simulink model "s_c107m32k_vlbi"  (R2018a)
settings: Solver=VariableStepDiscrete  StartTime=0.0  StopTime=(2^15)*10  RelTol=1e-3
undefined symbols (not defined in the file): fft_stages, n_bits_xengs
libraries: xbsIndex_r4 x23049, casper_library_misc x45, xps_library x4, casper_library_scopes x3, simulink x2
(part 29 of 201)

== system s_c107m32k_vlbi/quant_snap_filter1 ==
  note: This block filters out a single channel
      | from the quantiser so that if you want to get
      | a time-series of them in the snap instead of
      | a spectrum, you can do so.
  sync_in : Inport
  data_valid_in : Inport  Port=2
  data_in : Inport  Port=3
  packet_sync_in : Inport  Port=4
  single_channel_enable : Inport  Port=5
  channel_select : Inport  Port=6
  AddSub : xbsIndex_r4/AddSub  mode=Addition  use_carryin=off  use_carryout=off  en=off  latency=0  precision=User Defined  arith_type=Unsigned  n_bits=16  bin_pt=0  quantization=Truncate  overflow=Wrap  use_behavioral_HDL=off  hw_selection=Fabric  pipelined=off  dbl_ovrd=off  block_type=addsub
  Constant : xbsIndex_r4/Constant  const=4  gui_display_data_type=Fixed-point  arith_type=Unsigned  n_bits=3  bin_pt=0  preci_type=Single  exp_width=8  frac_width=24  explicit_period=on  period=1  equ=P=C  opselect=C  inp2=PCIN>>17  opr=+  inp1=P  carry=CIN  dbl_ovrd=off  block_type=constant
  Constant1 : xbsIndex_r4/Constant  const=0  gui_display_data_type=Fixed-point  arith_type=Unsigned  n_bits=3  bin_pt=0  preci_type=Single  exp_width=8  frac_width=24  explicit_period=on  period=1  equ=P=C  opselect=C  inp2=PCIN>>17  opr=+  inp1=P  carry=CIN  dbl_ovrd=off  block_type=constant
  Counter : xbsIndex_r4/Counter  cnt_type=Free Running  cnt_to=4095  operation=Up  start_count=0  cnt_by_val=4  arith_type=Unsigned  n_bits=fft_stages - 1  bin_pt=0  load_pin=off  rst=on  en=on  explicit_period=on  period=1  use_behavioral_HDL=off  implementation=Fabric  dbl_ovrd=off  block_type=counter
  Delay : xbsIndex_r4/Delay  rst=off  infoeditControl=Selection of Reset will increase slice count due to use of real FFs and instead of SRLs  en=off  latency=3  reg_retiming=off  dbl_ovrd=off  block_type=delay
  Delay{1..2,11..13} (5 alike) : xbsIndex_r4/Delay  rst=off  infoeditControl=Selection of Reset will increase slice count due to use of real FFs and instead of SRLs  en=off  latency=1  reg_retiming=off  dbl_ovrd=off  block_type=delay
  Delay{5,8..10} (4 alike) : xbsIndex_r4/Delay  rst=off  infoeditControl=Selection of Reset will increase slice count due to use of real FFs and instead of SRLs  en=off  latency=2  reg_retiming=off  dbl_ovrd=off  block_type=delay
  Logical1 : xbsIndex_r4/Logical  logical_function=AND  inputs=4  en=off  latency=0  precision=Full  arith_type=Unsigned  n_bits=16  bin_pt=0  align_bp=on  dbl_ovrd=off  block_type=logical
  Mux1 : xbsIndex_r4/Mux  inputs=2  en=off  latency=3  precision=Full  arith_type=Unsigned  n_bits=16  bin_pt=14  quantization=Truncate  overflow=Wrap  dbl_ovrd=off  block_type=mux
  Mux2 : xbsIndex_r4/Mux  inputs=2  en=off  latency=3  precision=Full  arith_type=Unsigned  n_bits=16  bin_pt=14  quantization=Truncate  overflow=Wrap  dbl_ovrd=off  block_type=mux
  Register : xbsIndex_r4/Register  init=0  rst=on  en=on  dbl_ovrd=off  block_type=register
  Register1 : xbsIndex_r4/Register  init=0  rst=on  en=on  dbl_ovrd=off  block_type=register
  Relational1 : xbsIndex_r4/Relational  mode=a>=b  op_type=Bool  en=off  latency=2  dbl_ovrd=off  block_type=relational
  Relational2 : xbsIndex_r4/Relational  mode=a<b  op_type=Bool  en=off  latency=2  dbl_ovrd=off  block_type=relational
  Relational3 : xbsIndex_r4/Relational  mode=a=b  op_type=Bool  en=off  latency=1  dbl_ovrd=off  block_type=relational
  edge_detect1 : Subsystem  mask(edge_detect){edge=Rising, polarity=Active High, x_in=[0 0.08 0.08 0.16 0.16 0.24 0.24 0.32 0.32 0.4], y_in=[-1 -1  1  1  1  1  1  1  1  1], x_out=[0.6 0.68 0.68 0.76 0.76 0.84 0.84 0.92 0.92 1], y_out=[-1 -1  1  1 -1 -1 -1 -1 -1 -1]}
      mask prompts: edge "Edge Type"; polarity "Output Polarity"; x_in "Input X Positions"; y_in "Input Y Positions"; x_out "Output X Positions"; y_out "Output Y Positions"
      mask help: Output is active for one-cycle after each edge of the specified type (i.e. rising, falling or both).
      mask init: same as s_c107m32k_vlbi/edge_detect1
      settings: AttributesFormatString=|
      | rising edges
      | active high
      mask Help: Output is active for one-cycle after each edge of the specified type (i.e. rising, falling, or both).  Latency is zero.
      mask TypeOptions edge: Rising | Falling | Both
      mask TypeOptions polarity: Active High | Active Low
      mask Display:
      | plot(x_in_num,0.5+y_in_num*0.2);
      | plot(x_out_num,0.5+y_out_num*0.2);
  edge_detect2 : Subsystem  mask(edge_detect){edge=Rising, polarity=Active High, x_in=[0 0.08 0.08 0.16 0.16 0.24 0.24 0.32 0.32 0.4], y_in=[-1 -1  1  1  1  1  1  1  1  1], x_out=[0.6 0.68 0.68 0.76 0.76 0.84 0.84 0.92 0.92 1], y_out=[-1 -1  1  1 -1 -1 -1 -1 -1 -1]}
      mask prompts: edge "Edge Type"; polarity "Output Polarity"; x_in "Input X Positions"; y_in "Input Y Positions"; x_out "Output X Positions"; y_out "Output Y Positions"
      mask help: Output is active for one-cycle after each edge of the specified type (i.e. rising, falling or both).
      mask init: same as s_c107m32k_vlbi/edge_detect1
      settings: AttributesFormatString=|
      | rising edges
      | active high
      mask Help: Output is active for one-cycle after each edge of the specified type (i.e. rising, falling, or both).  Latency is zero.
      mask TypeOptions edge: Rising | Falling | Both
      mask TypeOptions polarity: Active High | Active Low
      mask Display:
      | plot(x_in_num,0.5+y_in_num*0.2);
      | plot(x_out_num,0.5+y_out_num*0.2);
  edge_detect9 : Subsystem  mask(edge_detect){edge=Rising, polarity=Active High, x_in=[0 0.08 0.08 0.16 0.16 0.24 0.24 0.32 0.32 0.4], y_in=[-1 -1  1  1  1  1  1  1  1  1], x_out=[0.6 0.68 0.68 0.76 0.76 0.84 0.84 0.92 0.92 1], y_out=[-1 -1  1  1 -1 -1 -1 -1 -1 -1]}
      mask prompts: edge "Edge Type"; polarity "Output Polarity"; x_in "Input X Positions"; y_in "Input Y Positions"; x_out "Output X Positions"; y_out "Output Y Positions"
      mask help: Output is active for one-cycle after each edge of the specified type (i.e. rising, falling or both).
      mask init: same as s_c107m32k_vlbi/edge_detect1
      settings: AttributesFormatString=|
      | rising edges
      | active high
      mask Help: Output is active for one-cycle after each edge of the specified type (i.e. rising, falling, or both).  Latency is zero.
      mask TypeOptions edge: Rising | Falling | Both
      mask TypeOptions polarity: Active High | Active Low
      mask Display:
      | plot(x_in_num,0.5+y_in_num*0.2);
      | plot(x_out_num,0.5+y_out_num*0.2);
  data_valid_out : Outport
  data_out : Outport  Port=2
  packet_sync_out : Outport  Port=3
  wires:
  Delay13/1 -> Delay9/1
  Delay12/1 -> Delay8/1
  Delay11/1 -> Delay10/1, Delay2/1
  [packet_sync] -> Register1/3, Register1/1
  [sync_in] -> Register1/2
  Register1/1 -> edge_detect2/1(in)
  edge_detect2/1(out) -> Counter/1, Register/2
  Delay10/1 -> Mux2/2
  Delay9/1 -> Mux1/2
  Delay8/1 -> Delay/1
  edge_detect1/1(out) -> [selected_channel_active]
  edge_detect9/1(out) -> Mux2/3
  Logical1/1 -> edge_detect1/1(in)
  Delay5/1 -> Logical1/4
  Relational1/1 -> Logical1/3
  Relational2/1 -> Logical1/2
  Constant1/1 -> Relational3/1
  Relational3/1 -> edge_detect9/1(in)
  Counter/1 -> Relational3/2, AddSub/2, Relational1/2
  Delay2/1 -> Register/1, Register/3
  Register/1 -> Logical1/1
  AddSub/1 -> Relational2/2
  Constant/1 -> AddSub/1
  [packet_sync] -> Delay11/1
  Delay/1 -> data_out/1
  data_valid_in/1 -> [data_valid]
  Mux1/1 -> data_valid_out/1
  data_in/1 -> [data]
  [data_valid] -> Delay13/1
  sync_in/1 -> [sync_in]
  [selected_channel_active] -> Mux1/3
  packet_sync_in/1 -> [packet_sync]
  [data] -> Delay12/1
  [channel_select] -> Relational1/1, Relational2/1
  Mux2/1 -> packet_sync_out/1
  single_channel_enable/1 -> [single_channel_enable]
  [data_valid] -> Delay1/1
  [single_channel_enable] -> Mux1/1, Mux2/1
  channel_select/1 -> [channel_select]
  Delay1/1 -> Counter/2, Delay5/1

== system s_c107m32k_vlbi/quant_status ==
  out_pol0_or_cnt : Inport
  out_pol1_or_cnt : Inport  Port=2
  assert_pol0_or_cnt : xbsIndex_r4/Assert  assert_type=on  type_source=Explicitly  gui_display_data_type=Fixed-point  arith_type=Unsigned  n_bits=6  bin_pt=0  preci_type=Single  exp_width=8  frac_width=24  assert_rate=off  rate_source=Explicitly  period=1  output_port=on  block_type=assert
  assert_pol1_or_cnt : xbsIndex_r4/Assert  assert_type=on  type_source=Explicitly  gui_display_data_type=Fixed-point  arith_type=Unsigned  n_bits=6  bin_pt=0  preci_type=Single  exp_width=8  frac_width=24  assert_rate=off  rate_source=Explicitly  period=1  output_port=on  block_type=assert
  cast_gw : xbsIndex_r4/Convert  gui_display_data_type=Fixed-point  arith_type=Unsigned  n_bits=32  bin_pt=0  float_type=Single  exp_bits=8  fraction_bits=24  quantization=Truncate  overflow=Wrap  en=off  latency=1  pipeline=off  dbl_ovrd=off  block_type=convert
  concatenate : xbsIndex_r4/Concat  num_inputs=2  dbl_ovrd=off  block_type=concat
  io_delay : xbsIndex_r4/Delay  rst=off  infoeditControl=Selection of Reset will increase slice count due to use of real FFs and instead of SRLs  en=off  latency=0  reg_retiming=on  dbl_ovrd=off  block_type=delay
  reint1 : xbsIndex_r4/Reinterpret  force_arith_type=on  arith_type=Unsigned  force_bin_pt=on  bin_pt=0  block_type=reinterpret
  reint2 : xbsIndex_r4/Reinterpret  force_arith_type=on  arith_type=Unsigned  force_bin_pt=on  bin_pt=0  block_type=reinterpret
  s_c107m32k_vlbi_quant_status_user_data_in : xbsIndex_r4/Gateway Out  inherit_from_input=off  hdl_port=on  rows=1  columns=1  UseAsDAC=off  DACChannel='1'  interface=None  automatic_assignment=on  address_offset=hex2dec('00')  intf_name=''  intf_description=''  timing_constraint=None  locs_specified=off  LOCs={}  io_standard={}  block_type=gatewayout
  sim_out : Terminator
  wires:
  concatenate/1 -> io_delay/1
  io_delay/1 -> cast_gw/1
  cast_gw/1 -> s_c107m32k_vlbi_quant_status_user_data_in/1
  s_c107m32k_vlbi_quant_status_user_data_in/1 -> sim_out/1
  out_pol0_or_cnt/1 -> assert_pol0_or_cnt/1
  assert_pol0_or_cnt/1 -> reint1/1
  reint1/1 -> concatenate/1
  out_pol1_or_cnt/1 -> assert_pol1_or_cnt/1
  assert_pol1_or_cnt/1 -> reint2/1
  reint2/1 -> concatenate/2

== system s_c107m32k_vlbi/quant_sync_cnt ==
  out_reg : Inport
  assert_reg : xbsIndex_r4/Assert  assert_type=on  type_source=Explicitly  gui_display_data_type=Fixed-point  arith_type=Unsigned  n_bits=11  bin_pt=0  preci_type=Single  exp_width=8  frac_width=24  assert_rate=off  rate_source=Explicitly  period=1  output_port=on  block_type=assert
  cast_gw : xbsIndex_r4/Convert  gui_display_data_type=Fixed-point  arith_type=Unsigned  n_bits=32  bin_pt=0  float_type=Single  exp_bits=8  fraction_bits=24  quantization=Truncate  overflow=Wrap  en=off  latency=1  pipeline=off  dbl_ovrd=off  block_type=convert
  io_delay : xbsIndex_r4/Delay  rst=off  infoeditControl=Selection of Reset will increase slice count due to use of real FFs and instead of SRLs  en=off  latency=0  reg_retiming=on  dbl_ovrd=off  block_type=delay
  reint1 : xbsIndex_r4/Reinterpret  force_arith_type=on  arith_type=Unsigned  force_bin_pt=on  bin_pt=0  block_type=reinterpret
  s_c107m32k_vlbi_quant_sync_cnt_user_data_in : xbsIndex_r4/Gateway Out  inherit_from_input=off  hdl_port=on  rows=1  columns=1  UseAsDAC=off  DACChannel='1'  interface=None  automatic_assignment=on  address_offset=hex2dec('00')  intf_name=''  intf_description=''  timing_constraint=None  locs_specified=off  LOCs={}  io_standard={}  block_type=gatewayout
  sim_out : Terminator
  wires:
  io_delay/1 -> cast_gw/1
  cast_gw/1 -> s_c107m32k_vlbi_quant_sync_cnt_user_data_in/1
  s_c107m32k_vlbi_quant_sync_cnt_user_data_in/1 -> sim_out/1
  out_reg/1 -> assert_reg/1
  assert_reg/1 -> reint1/1
  reint1/1 -> io_delay/1

== system s_c107m32k_vlbi/reorder_status ==
  out_timestep_err_cnt : Inport
  out_receive_err_cnt : Inport  Port=2
  out_discard_cnt : Inport  Port=3
  out_relock_err_cnt : Inport  Port=4
  out_overflow_err_cnt : Inport  Port=5
  out_dv_cnt : Inport  Port=6
  assert_discard_cnt : xbsIndex_r4/Assert  assert_type=on  type_source=Explicitly  gui_display_data_type=Fixed-point  arith_type=Unsigned  n_bits=5  bin_pt=0  preci_type=Single  exp_width=8  frac_width=24  assert_rate=off  rate_source=Explicitly  period=1  output_port=on  block_type=assert
  assert_dv_cnt : xbsIndex_r4/Assert  assert_type=on  type_source=Explicitly  gui_display_data_type=Fixed-point  arith_type=Unsigned  n_bits=5  bin_pt=0  preci_type=Single  exp_width=8  frac_width=24  assert_rate=off  rate_source=Explicitly  period=1  output_port=on  block_type=assert
  assert_overflow_err_cnt : xbsIndex_r4/Assert  assert_type=on  type_source=Explicitly  gui_display_data_type=Fixed-point  arith_type=Unsigned  n_bits=5  bin_pt=0  preci_type=Single  exp_width=8  frac_width=24  assert_rate=off  rate_source=Explicitly  period=1  output_port=on  block_type=assert
  assert_receive_err_cnt : xbsIndex_r4/Assert  assert_type=on  type_source=Explicitly  gui_display_data_type=Fixed-point  arith_type=Unsigned  n_bits=5  bin_pt=0  preci_type=Single  exp_width=8  frac_width=24  assert_rate=off  rate_source=Explicitly  period=1  output_port=on  block_type=assert
  assert_relock_err_cnt : xbsIndex_r4/Assert  assert_type=on  type_source=Explicitly  gui_display_data_type=Fixed-point  arith_type=Unsigned  n_bits=5  bin_pt=0  preci_type=Single  exp_width=8  frac_width=24  assert_rate=off  rate_source=Explicitly  period=1  output_port=on  block_type=assert
  assert_timestep_err_cnt : xbsIndex_r4/Assert  assert_type=on  type_source=Explicitly  gui_display_data_type=Fixed-point  arith_type=Unsigned  n_bits=5  bin_pt=0  preci_type=Single  exp_width=8  frac_width=24  assert_rate=off  rate_source=Explicitly  period=1  output_port=on  block_type=assert
  cast_gw : xbsIndex_r4/Convert  gui_display_data_type=Fixed-point  arith_type=Unsigned  n_bits=32  bin_pt=0  float_type=Single  exp_bits=8  fraction_bits=24  quantization=Truncate  overflow=Wrap  en=off  latency=1  pipeline=off  dbl_ovrd=off  block_type=convert
  concatenate : xbsIndex_r4/Concat  num_inputs=6  dbl_ovrd=off  block_type=concat
  io_delay : xbsIndex_r4/Delay  rst=off  infoeditControl=Selection of Reset will increase slice count due to use of real FFs and instead of SRLs  en=off  latency=0  reg_retiming=on  dbl_ovrd=off  block_type=delay
  reint{1..6} (6 alike) : xbsIndex_r4/Reinterpret  force_arith_type=on  arith_type=Unsigned  force_bin_pt=on  bin_pt=0  block_type=reinterpret
  s_c107m32k_vlbi_reorder_status_user_data_in : xbsIndex_r4/Gateway Out  inherit_from_input=off  hdl_port=on  rows=1  columns=1  UseAsDAC=off  DACChannel='1'  interface=None  automatic_assignment=on  address_offset=hex2dec('00')  intf_name=''  intf_description=''  timing_constraint=None  locs_specified=off  LOCs={}  io_standard={}  block_type=gatewayout
  sim_out : Terminator
  wires:
  concatenate/1 -> io_delay/1
  io_delay/1 -> cast_gw/1
  cast_gw/1 -> s_c107m32k_vlbi_reorder_status_user_data_in/1
  s_c107m32k_vlbi_reorder_status_user_data_in/1 -> sim_out/1
  out_timestep_err_cnt/1 -> assert_timestep_err_cnt/1
  assert_timestep_err_cnt/1 -> reint1/1
  reint1/1 -> concatenate/1
  out_receive_err_cnt/1 -> assert_receive_err_cnt/1
  assert_receive_err_cnt/1 -> reint2/1
  reint2/1 -> concatenate/2
  out_discard_cnt/1 -> assert_discard_cnt/1
  assert_discard_cnt/1 -> reint3/1
  reint3/1 -> concatenate/3
  out_relock_err_cnt/1 -> assert_relock_err_cnt/1
  assert_relock_err_cnt/1 -> reint4/1
  reint4/1 -> concatenate/4
  out_overflow_err_cnt/1 -> assert_overflow_err_cnt/1
  assert_overflow_err_cnt/1 -> reint5/1
  reint5/1 -> concatenate/5
  out_dv_cnt/1 -> assert_dv_cnt/1
  assert_dv_cnt/1 -> reint6/1
  reint6/1 -> concatenate/6

== system s_c107m32k_vlbi/reorder_status1 ==
  out_dv_per_sec : Inport
  assert_dv_per_sec : xbsIndex_r4/Assert  assert_type=on  type_source=Explicitly  gui_display_data_type=Fixed-point  arith_type=Unsigned  n_bits=32  bin_pt=0  preci_type=Single  exp_width=8  frac_width=24  assert_rate=off  rate_source=Explicitly  period=1  output_port=on  block_type=assert
  cast_gw : xbsIndex_r4/Convert  gui_display_data_type=Fixed-point  arith_type=Unsigned  n_bits=32  bin_pt=0  float_type=Single  exp_bits=8  fraction_bits=24  quantization=Truncate  overflow=Wrap  en=off  latency=1  pipeline=off  dbl_ovrd=off  block_type=convert
  io_delay : xbsIndex_r4/Delay  rst=off  infoeditControl=Selection of Reset will increase slice count due to use of real FFs and instead of SRLs  en=off  latency=0  reg_retiming=on  dbl_ovrd=off  block_type=delay
  reint1 : xbsIndex_r4/Reinterpret  force_arith_type=on  arith_type=Unsigned  force_bin_pt=on  bin_pt=0  block_type=reinterpret
  s_c107m32k_vlbi_reorder_status1_user_data_in : xbsIndex_r4/Gateway Out  inherit_from_input=off  hdl_port=on  rows=1  columns=1  UseAsDAC=off  DACChannel='1'  interface=None  automatic_assignment=on  address_offset=hex2dec('00')  intf_name=''  intf_description=''  timing_constraint=None  locs_specified=off  LOCs={}  io_standard={}  block_type=gatewayout
  sim_out : Terminator
  wires:
  io_delay/1 -> cast_gw/1
  cast_gw/1 -> s_c107m32k_vlbi_reorder_status1_user_data_in/1
  s_c107m32k_vlbi_reorder_status1_user_data_in/1 -> sim_out/1
  out_dv_per_sec/1 -> assert_dv_per_sec/1
  assert_dv_per_sec/1 -> reint1/1
  reint1/1 -> io_delay/1

== system s_c107m32k_vlbi/rx_dest_ip ==
  out_reg : Inport
  assert_reg : xbsIndex_r4/Assert  assert_type=on  type_source=Explicitly  gui_display_data_type=Fixed-point  arith_type=Unsigned  n_bits=32  bin_pt=0  preci_type=Single  exp_width=8  frac_width=24  assert_rate=off  rate_source=Explicitly  period=1  output_port=on  block_type=assert
  cast_gw : xbsIndex_r4/Convert  gui_display_data_type=Fixed-point  arith_type=Unsigned  n_bits=32  bin_pt=0  float_type=Single  exp_bits=8  fraction_bits=24  quantization=Truncate  overflow=Wrap  en=off  latency=1  pipeline=off  dbl_ovrd=off  block_type=convert
  io_delay : xbsIndex_r4/Delay  rst=off  infoeditControl=Selection of Reset will increase slice count due to use of real FFs and instead of SRLs  en=off  latency=0  reg_retiming=on  dbl_ovrd=off  block_type=delay
  reint1 : xbsIndex_r4/Reinterpret  force_arith_type=on  arith_type=Unsigned  force_bin_pt=on  bin_pt=0  block_type=reinterpret
  s_c107m32k_vlbi_rx_dest_ip_user_data_in : xbsIndex_r4/Gateway Out  inherit_from_input=off  hdl_port=on  rows=1  columns=1  UseAsDAC=off  DACChannel='1'  interface=None  automatic_assignment=on  address_offset=hex2dec('00')  intf_name=''  intf_description=''  timing_constraint=None  locs_specified=off  LOCs={}  io_standard={}  block_type=gatewayout
  sim_out : Terminator
  wires:
  io_delay/1 -> cast_gw/1
  cast_gw/1 -> s_c107m32k_vlbi_rx_dest_ip_user_data_in/1
  s_c107m32k_vlbi_rx_dest_ip_user_data_in/1 -> sim_out/1
  out_reg/1 -> assert_reg/1
  assert_reg/1 -> reint1/1
  reint1/1 -> io_delay/1

== system s_c107m32k_vlbi/simple_bram_vacc1 ==
  new_acc : Inport
  din : Inport  Port=2
  dvalid : Inport  Port=3
  Adder : xbsIndex_r4/AddSub  mode=Addition  use_carryin=off  use_carryout=off  en=on  latency=2  precision=User Defined  arith_type=Unsigned  n_bits=n_bits  bin_pt=bin_pt  quantization=Truncate  overflow=Wrap  use_behavioral_HDL=on  hw_selection=Fabric  pipelined=off  use_rpm=on  dbl_ovrd=off  block_type=addsub
      settings: xl_area=[0, 0, 0, 0, 0, 0, 0]  block_version=10.1.3
  Constant : xbsIndex_r4/Constant  const=0  gui_display_data_type=Fixed-point  arith_type=Unsigned  n_bits=n_bits  bin_pt=bin_pt  preci_type=Single  exp_width=8  frac_width=24  explicit_period=on  period=1  equ=P=C  opselect=C  inp2=PCIN>>17  opr=+  inp1=P  carry=CIN  dbl_ovrd=off  block_type=constant
  Delay17 : xbsIndex_r4/Delay  rst=off  infoeditControl=Selection of Reset will increase slice count due to use of real FFs and instead of SRLs  en=off  latency=1  reg_retiming=on  dbl_ovrd=off  block_type=delay
  Gateway Out{1..3,71} (4 alike) : xbsIndex_r4/Gateway Out  inherit_from_input=off  hdl_port=off  rows=1  columns=1  UseAsDAC=off  DACChannel='1'  interface=None  automatic_assignment=on  address_offset=hex2dec('00')  intf_name=''  intf_description=''  timing_constraint=None  locs_specified=off  LOCs={}  io_standard={}  block_type=gatewayout
  Logical : xbsIndex_r4/Logical  logical_function=AND  inputs=2  en=off  latency=0  precision=Full  arith_type=Unsigned  n_bits=16  bin_pt=0  align_bp=on  dbl_ovrd=off  block_type=logical
  Mux : xbsIndex_r4/Mux  inputs=2  en=off  latency=0  precision=Full  arith_type="Signed  (2's comp)"  n_bits=8  bin_pt=2  quantization=Truncate  overflow=Wrap  dbl_ovrd=off  block_type=mux
      settings: xl_area=[0, 0, 0, 0, 0, 0, 0]
  To Workspace1 : ToWorkspace  VariableName=tp28  SaveFormat=Timeseries  SampleTime=-1
  To Workspace2 : ToWorkspace  VariableName=tp29  SaveFormat=Timeseries  SampleTime=-1
  To Workspace3 : ToWorkspace  VariableName=tp30  SaveFormat=Timeseries  SampleTime=-1
  To Workspace71 : ToWorkspace  VariableName=tp27  SaveFormat=Timeseries  SampleTime=-1
  delay_bram : Subsystem  mask(delay_bram){DelayLen=vec_len - 2, bram_latency=2}
      mask prompts: DelayLen "Delay By:"; bram_latency "BRAM Latency"
      mask help: A delay block that uses BRAM for its storage.
      mask init:
      | if (DelayLen <= bram_latency)
      | 	error('delay value must be greater than BRAM Latency');
      | end
      | BitWidth = max(ceil(log2(DelayLen)), 2);
      mask Help: eval('xlWeb(''http://casper.berkeley.edu/wiki/Delay_bram'')')
  pulse_ext : Subsystem  mask(pulse_ext){pulse_len=vec_len}
      mask prompts: pulse_len "Length of Pulse"
      mask help:
      | Extends a boolean signal to be high for the specified number of clocks after
      | the last high input.
      mask init:
      | bits = ceil(log2(pulse_len+1));
      mask Help: eval('xlWeb(''http://casper.berkeley.edu/wiki/Pulse_ext'')')
  dout : Outport
  valid : Outport  Port=2
  wires:
  delay_bram/1(Out1) -> Gateway Out3/1, dout/1, Mux/2
  new_acc/1 -> pulse_ext/1(in)
  Constant/1 -> Mux/3
  din/1 -> Adder/1
  Adder/1 -> delay_bram/1(In1)
  pulse_ext/1(out) -> Gateway Out1/1, Logical/2, Mux/1
  dvalid/1 -> delay_bram/2(In2), Adder/3, Gateway Out71/1, Logical/1, pulse_ext/2(dvalid)
  Mux/1 -> Adder/2
  Logical/1 -> Delay17/1
  Gateway Out71/1 -> To Workspace71/1
  Gateway Out1/1 -> To Workspace1/1
  Gateway Out2/1 -> To Workspace2/1
  Gateway Out3/1 -> To Workspace3/1
  Delay17/1 -> Gateway Out2/1, valid/1

== system s_c107m32k_vlbi/simple_bram_vacc2 ==
  new_acc : Inport
  din : Inport  Port=2
  dvalid : Inport  Port=3
  Adder : xbsIndex_r4/AddSub  mode=Addition  use_carryin=off  use_carryout=off  en=on  latency=2  precision=User Defined  arith_type=Unsigned  n_bits=n_bits  bin_pt=bin_pt  quantization=Truncate  overflow=Wrap  use_behavioral_HDL=on  hw_selection=Fabric  pipelined=off  use_rpm=on  dbl_ovrd=off  block_type=addsub
      settings: xl_area=[0, 0, 0, 0, 0, 0, 0]  block_version=10.1.3
  Constant : xbsIndex_r4/Constant  const=0  gui_display_data_type=Fixed-point  arith_type=Unsigned  n_bits=n_bits  bin_pt=bin_pt  preci_type=Single  exp_width=8  frac_width=24  explicit_period=on  period=1  equ=P=C  opselect=C  inp2=PCIN>>17  opr=+  inp1=P  carry=CIN  dbl_ovrd=off  block_type=constant
  Delay17 : xbsIndex_r4/Delay  rst=off  infoeditControl=Selection of Reset will increase slice count due to use of real FFs and instead of SRLs  en=off  latency=2  reg_retiming=on  dbl_ovrd=off  block_type=delay
  Gateway Out{1..3,71} (4 alike) : xbsIndex_r4/Gateway Out  inherit_from_input=off  hdl_port=off  rows=1  columns=1  UseAsDAC=off  DACChannel='1'  interface=None  automatic_assignment=on  address_offset=hex2dec('00')  intf_name=''  intf_description=''  timing_constraint=None  locs_specified=off  LOCs={}  io_standard={}  block_type=gatewayout
  Logical : xbsIndex_r4/Logical  logical_function=AND  inputs=2  en=off  latency=0  precision=Full  arith_type=Unsigned  n_bits=16  bin_pt=0  align_bp=on  dbl_ovrd=off  block_type=logical
  Mux : xbsIndex_r4/Mux  inputs=2  en=off  latency=0  precision=Full  arith_type="Signed  (2's comp)"  n_bits=8  bin_pt=2  quantization=Truncate  overflow=Wrap  dbl_ovrd=off  block_type=mux
      settings: xl_area=[0, 0, 0, 0, 0, 0, 0]
  To Workspace1 : ToWorkspace  VariableName=tp28  SaveFormat=Timeseries  SampleTime=-1
  To Workspace2 : ToWorkspace  VariableName=tp29  SaveFormat=Timeseries  SampleTime=-1
  To Workspace3 : ToWorkspace  VariableName=tp30  SaveFormat=Timeseries  SampleTime=-1
  To Workspace71 : ToWorkspace  VariableName=tp27  SaveFormat=Timeseries  SampleTime=-1
  delay_bram : Subsystem  mask(delay_bram){DelayLen=vec_len - 2, bram_latency=2}
      mask prompts: DelayLen "Delay By:"; bram_latency "BRAM Latency"
      mask help: A delay block that uses BRAM for its storage.
      mask init:
      | if (DelayLen <= bram_latency)
      | 	error('delay value must be greater than BRAM Latency');
      | end
      | BitWidth = max(ceil(log2(DelayLen)), 2);
      mask Help: eval('xlWeb(''http://casper.berkeley.edu/wiki/Delay_bram'')')
  pulse_ext : Subsystem  mask(pulse_ext){pulse_len=vec_len}
      mask prompts: pulse_len "Length of Pulse"
      mask help:
      | Extends a boolean signal to be high for the specified number of clocks after
      | the last high input.
      mask init:
      | bits = ceil(log2(pulse_len+1));
      mask Help: eval('xlWeb(''http://casper.berkeley.edu/wiki/Pulse_ext'')')
  dout : Outport
  valid : Outport  Port=2
  wires:
  Delay17/1 -> valid/1, Gateway Out2/1
  Gateway Out3/1 -> To Workspace3/1
  Gateway Out2/1 -> To Workspace2/1
  Gateway Out1/1 -> To Workspace1/1
  Gateway Out71/1 -> To Workspace71/1
  Logical/1 -> Delay17/1
  Mux/1 -> Adder/2
  dvalid/1 -> pulse_ext/2(dvalid), Logical/1, Gateway Out71/1, Adder/3, delay_bram/2(In2)
  pulse_ext/1(out) -> Mux/1, Logical/2, Gateway Out1/1
  Adder/1 -> delay_bram/1(In1)
  din/1 -> Adder/1
  Constant/1 -> Mux/3
  new_acc/1 -> pulse_ext/1(in)
  delay_bram/1(Out1) -> Mux/2, dout/1, Gateway Out3/1

== system s_c107m32k_vlbi/snap_acc ==
  in_acc : Inport
  we : Inport  Port=2
  trig : Inport  Port=3
  assert_acc : xbsIndex_r4/Assert  assert_type=on  type_source=Explicitly  gui_display_data_type=Fixed-point  arith_type=Unsigned  n_bits=32  bin_pt=10  preci_type=Single  exp_width=8  frac_width=24  assert_rate=off  rate_source=Explicitly  period=1  output_port=on  block_type=assert
  buscreate : Subsystem  AncestorBlock=casper_library_flow_control/bus_create  mask(bus_create){inputNum=1}
      mask prompts: inputNum "Number of inputs:"
      mask init:
      | bus_create_init(gcb,...
      |     'inputNum', inputNum);
  io_delay : Subsystem  AncestorBlock=casper_library_delays/pipeline  mask(pipeline){csp_latency=2}
      mask prompts: csp_latency "Latency"
      mask help:
      | An explicitly laid-out delay line to avoid mapping to SRL16s
      | for use in pipelining to help achieve timing closure.
      mask init:
      | pipeline_init(gcb,'latency',csp_latency);
      settings: AttributesFormatString=Latency = %<latency>
      mask Display:
      | port_label('input', 1, 'd');
      | port_label('output', 1, 'q');
      | disp(['Z^-', num2str(csp_latency)]);
  ss : Subsystem  Tag=casper:snapshot  AncestorBlock=casper_library_scopes/snapshot  mask(snapshot){storage=bram, dram_dimm=2, dram_clock=250, nsamples=15, data_width=32, offset=off, circap=off, value=off, ext_arm=off, ext_circ=off, provide_outputs=off, use_dsp48=on}
      mask prompts: storage "Storage medium"; dram_dimm "DRAM dimm"; dram_clock "DRAM clock rate"; nsamples "Number of Samples (2^?)"; data_width "Data width"; offset "Start delay support"; circap "Circular capture support"; value "Extra value capture support"; ext_arm "External arm support"; ext_circ "External circular capture support"; provide_outputs "Provide outputs"; use_dsp48 "Use DSP48s to implement counters"
      mask help:
      | Standard snap block, but with the following optional extras;
      |  1) Optionally delay the fabric trigger by a user-specified number of valids.
      |  2) Capture continuously after a trigger until a stop pulse is received. Data is captured into BRAM continuously, with old data being overwritten until a stop command is received. Then stop capturing when memory is filled. This enables you to get some data before and some data after the stop pulse. Use the 'tr_en_cnt' register to determine where you are in your vector. 'Addr' register's MSb now indicates 'busy capturing'.
      |  3) Optionally capture a value on an input port to a register at the same time as the first data sample.
      |  4) Implement counters using DSP48Es to save resources.
      mask init:
      | snapshot_init(gcb, ...
      |     'storage', storage, ...
      |     'dram_dimm', dram_dimm, ...
      |     'dram_clock', dram_clock, ...
      |     'nsamples', nsamples, ...
      |     'data_width', data_width, ...
      |     'offset', offset, ...
      |     'circap', circap, ...
      |     'value', value, ...
      |     'ext_arm', ext_arm, ...
      |     'ext_circ', ext_circ, ...
      |     'provide_outputs', 'off', ...
      |     'use_dsp48', use_dsp48);
      settings: AttributesFormatString=|
      | 32 wide, 32768 deep
      | debugID: 110166481
      mask TypeOptions storage: bram | dram
      mask Callback storage: snapshot_callback();
      mask TypeOptions dram_dimm: 1 | 2 | 3 | 4
      mask TypeOptions dram_clock: 200 | 250 | 266 | 300 | 333
      mask TypeOptions data_width: 8 | 16 | 32 | 64 | 128
  trig_delay : Subsystem  AncestorBlock=casper_library_delays/pipeline  mask(pipeline){csp_latency=2}
      mask prompts: csp_latency "Latency"
      mask help:
      | An explicitly laid-out delay line to avoid mapping to SRL16s
      | for use in pipelining to help achieve timing closure.
      mask init:
      | pipeline_init(gcb,'latency',csp_latency);
      settings: AttributesFormatString=Latency = %<latency>
      mask Display:
      | port_label('input', 1, 'd');
      | port_label('output', 1, 'q');
      | disp(['Z^-', num2str(csp_latency)]);
  we_delay : Subsystem  AncestorBlock=casper_library_delays/pipeline  mask(pipeline){csp_latency=2}
      mask prompts: csp_latency "Latency"
      mask help:
      | An explicitly laid-out delay line to avoid mapping to SRL16s
      | for use in pipelining to help achieve timing closure.
      mask init:
      | pipeline_init(gcb,'latency',csp_latency);
      settings: AttributesFormatString=Latency = %<latency>
      mask Display:
      | port_label('input', 1, 'd');
      | port_label('output', 1, 'q');
      | disp(['Z^-', num2str(csp_latency)]);
  arm_out : Outport
  wires:
  ss/1(arm_out) -> arm_out/1
  buscreate/1(bus_out) -> io_delay/1(d)
  io_delay/1(q) -> ss/1(din)
  in_acc/1 -> assert_acc/1
  assert_acc/1 -> buscreate/1(in1)
  we/1 -> we_delay/1(d)
  we_delay/1(q) -> ss/2(we)
  trig/1 -> trig_delay/1(d)
  trig_delay/1(q) -> ss/3(trig)

== system s_c107m32k_vlbi/snap_adc0 ==
  in_p0_d0 : Inport
  in_p0_d1 : Inport  Port=2
  in_p0_d2 : Inport  Port=3
  in_p0_d3 : Inport  Port=4
  in_p0_d4 : Inport  Port=5
  in_p0_d5 : Inport  Port=6
  in_p0_d6 : Inport  Port=7
  in_p0_d7 : Inport  Port=8
  in_dv : Inport  Port=9
  in_sync : Inport  Port=10
  we : Inport  Port=11
  trig : Inport  Port=12
  stop : Inport  Port=13
  extra_timestamp : Inport  Port=14
  assert_dv : xbsIndex_r4/Assert  assert_type=on  type_source=Explicitly  gui_display_data_type=Boolean  arith_type=Boolean  n_bits=1  bin_pt=0  preci_type=Single  exp_width=8  frac_width=24  assert_rate=off  rate_source=Explicitly  period=1  output_port=on  block_type=assert
  assert_p0_d{0..7} (8 alike) : xbsIndex_r4/Assert  assert_type=on  type_source=Explicitly  gui_display_data_type=Fixed-point  arith_type="Signed  (2's comp)"  n_bits=10  bin_pt=9  preci_type=Single  exp_width=8  frac_width=24  assert_rate=off  rate_source=Explicitly  period=1  output_port=on  block_type=assert
  assert_sync : xbsIndex_r4/Assert  assert_type=on  type_source=Explicitly  gui_display_data_type=Boolean  arith_type=Boolean  n_bits=1  bin_pt=0  preci_type=Single  exp_width=8  frac_width=24  assert_rate=off  rate_source=Explicitly  period=1  output_port=on  block_type=assert
  assextra_timestamp : xbsIndex_r4/Assert  assert_type=on  type_source=Explicitly  gui_display_data_type=Fixed-point  arith_type=Unsigned  n_bits=32  bin_pt=0  preci_type=Single  exp_width=8  frac_width=24  assert_rate=off  rate_source=Explicitly  period=1  output_port=on  block_type=assert
  buscreate : Subsystem  AncestorBlock=casper_library_flow_control/bus_create  mask(bus_create){inputNum=10}
      mask prompts: inputNum "Number of inputs:"
      mask init:
      | bus_create_init(gcb,...
      |     'inputNum', inputNum);
  extra_delay : Subsystem  AncestorBlock=casper_library_delays/pipeline  mask(pipeline){csp_latency=2}
      mask prompts: csp_latency "Latency"
      mask help:
      | An explicitly laid-out delay line to avoid mapping to SRL16s
      | for use in pipelining to help achieve timing closure.
      mask init:
      | pipeline_init(gcb,'latency',csp_latency);
      settings: AttributesFormatString=Latency = %<latency>
      mask Display:
      | port_label('input', 1, 'd');
      | port_label('output', 1, 'q');
      | disp(['Z^-', num2str(csp_latency)]);
  extracast : xbsIndex_r4/Convert  gui_display_data_type=Fixed-point  arith_type=Unsigned  n_bits=32  bin_pt=0  float_type=Single  exp_bits=8  fraction_bits=24  quantization=Truncate  overflow=Wrap  en=off  latency=1  pipeline=off  dbl_ovrd=off  block_type=convert
  extracreate : Subsystem  AncestorBlock=casper_library_flow_control/bus_create  mask(bus_create){inputNum=1}
      mask prompts: inputNum "Number of inputs:"
      mask init:
      | bus_create_init(gcb,...
      |     'inputNum', inputNum);
  io_delay : Subsystem  AncestorBlock=casper_library_delays/pipeline  mask(pipeline){csp_latency=2}
      mask prompts: csp_latency "Latency"
      mask help:
      | An explicitly laid-out delay line to avoid mapping to SRL16s
      | for use in pipelining to help achieve timing closure.
      mask init:
      | pipeline_init(gcb,'latency',csp_latency);
      settings: AttributesFormatString=Latency = %<latency>
      mask Display:
      | port_label('input', 1, 'd');
      | port_label('output', 1, 'q');
      | disp(['Z^-', num2str(csp_latency)]);
  ss : Subsystem  Tag=casper:snapshot  AncestorBlock=casper_library_scopes/snapshot  mask(snapshot){storage=bram, dram_dimm=2, dram_clock=250, nsamples=8, data_width=128, offset=off, circap=on, value=on, ext_arm=off, ext_circ=off, provide_outputs=off, use_dsp48=on}
      mask prompts: storage "Storage medium"; dram_dimm "DRAM dimm"; dram_clock "DRAM clock rate"; nsamples "Number of Samples (2^?)"; data_width "Data width"; offset "Start delay support"; circap "Circular capture support"; value "Extra value capture support"; ext_arm "External arm support"; ext_circ "External circular capture support"; provide_outputs "Provide outputs"; use_dsp48 "Use DSP48s to implement counters"
      mask help:
      | Standard snap block, but with the following optional extras;
      |  1) Optionally delay the fabric trigger by a user-specified number of valids.
      |  2) Capture continuously after a trigger until a stop pulse is received. Data is captured into BRAM continuously, with old data being overwritten until a stop command is received. Then stop capturing when memory is filled. This enables you to get some data before and some data after the stop pulse. Use the 'tr_en_cnt' register to determine where you are in your vector. 'Addr' register's MSb now indicates 'busy capturing'.
      |  3) Optionally capture a value on an input port to a register at the same time as the first data sample.
      |  4) Implement counters using DSP48Es to save resources.
      mask init: same as s_c107m32k_vlbi/snap_acc/ss
      settings: AttributesFormatString=|
      | 128 wide, 256 deep
      | debugID: 56897180
      mask TypeOptions storage: bram | dram
      mask Callback storage: snapshot_callback();
      mask TypeOptions dram_dimm: 1 | 2 | 3 | 4
      mask TypeOptions dram_clock: 200 | 250 | 266 | 300 | 333
      mask TypeOptions data_width: 8 | 16 | 32 | 64 | 128
  stop_delay : Subsystem  AncestorBlock=casper_library_delays/pipeline  mask(pipeline){csp_latency=2}
      mask prompts: csp_latency "Latency"
      mask help:
      | An explicitly laid-out delay line to avoid mapping to SRL16s
      | for use in pipelining to help achieve timing closure.
      mask init:
      | pipeline_init(gcb,'latency',csp_latency);
      settings: AttributesFormatString=Latency = %<latency>
      mask Display:
      | port_label('input', 1, 'd');
      | port_label('output', 1, 'q');
      | disp(['Z^-', num2str(csp_latency)]);
  trig_delay : Subsystem  AncestorBlock=casper_library_delays/pipeline  mask(pipeline){csp_latency=2}
      mask prompts: csp_latency "Latency"
      mask help:
      | An explicitly laid-out delay line to avoid mapping to SRL16s
      | for use in pipelining to help achieve timing closure.
      mask init:
      | pipeline_init(gcb,'latency',csp_latency);
      settings: AttributesFormatString=Latency = %<latency>
      mask Display:
      | port_label('input', 1, 'd');
      | port_label('output', 1, 'q');
      | disp(['Z^-', num2str(csp_latency)]);
  we_delay : Subsystem  AncestorBlock=casper_library_delays/pipeline  mask(pipeline){csp_latency=2}
      mask prompts: csp_latency "Latency"
      mask help:
      | An explicitly laid-out delay line to avoid mapping to SRL16s
      | for use in pipelining to help achieve timing closure.
      mask init:
      | pipeline_init(gcb,'latency',csp_latency);
      settings: AttributesFormatString=Latency = %<latency>
      mask Display:
      | port_label('input', 1, 'd');
      | port_label('output', 1, 'q');
      | disp(['Z^-', num2str(csp_latency)]);
  arm_out : Outport
  wires:
  ss/1(arm_out) -> arm_out/1
  buscreate/1(bus_out) -> io_delay/1(d)
  io_delay/1(q) -> ss/1(din)
  in_p0_d0/1 -> assert_p0_d0/1
  assert_p0_d0/1 -> buscreate/1(in1)
  in_p0_d1/1 -> assert_p0_d1/1
  assert_p0_d1/1 -> buscreate/2(in2)
  in_p0_d2/1 -> assert_p0_d2/1
  assert_p0_d2/1 -> buscreate/3(in3)
  in_p0_d3/1 -> assert_p0_d3/1
  assert_p0_d3/1 -> buscreate/4(in4)
  in_p0_d4/1 -> assert_p0_d4/1
  assert_p0_d4/1 -> buscreate/5(in5)
  in_p0_d5/1 -> assert_p0_d5/1
  assert_p0_d5/1 -> buscreate/6(in6)
  in_p0_d6/1 -> assert_p0_d6/1
  assert_p0_d6/1 -> buscreate/7(in7)
  in_p0_d7/1 -> assert_p0_d7/1
  assert_p0_d7/1 -> buscreate/8(in8)
  in_dv/1 -> assert_dv/1
  assert_dv/1 -> buscreate/9(in9)
  in_sync/1 -> assert_sync/1
  assert_sync/1 -> buscreate/10(in10)
  we/1 -> we_delay/1(d)
  we_delay/1(q) -> ss/2(we)
  trig/1 -> trig_delay/1(d)
  trig_delay/1(q) -> ss/3(trig)
  stop/1 -> stop_delay/1(d)
  stop_delay/1(q) -> ss/4(stop)
  extracreate/1(bus_out) -> extra_delay/1(d)
  extra_delay/1(q) -> extracast/1
  extracast/1 -> ss/5(vin)
  extra_timestamp/1 -> assextra_timestamp/1
  assextra_timestamp/1 -> extracreate/1(in1)

== system s_c107m32k_vlbi/snap_adc1 ==
  in_p1_d0 : Inport
  in_p1_d1 : Inport  Port=2
  in_p1_d2 : Inport  Port=3
  in_p1_d3 : Inport  Port=4
  in_p1_d4 : Inport  Port=5
  in_p1_d5 : Inport  Port=6
  in_p1_d6 : Inport  Port=7
  in_p1_d7 : Inport  Port=8
  we : Inport  Port=9
  trig : Inport  Port=10
  stop : Inport  Port=11
  extra_timestamp : Inport  Port=12
  assert_p1_d{0..7} (8 alike) : xbsIndex_r4/Assert  assert_type=on  type_source=Explicitly  gui_display_data_type=Fixed-point  arith_type="Signed  (2's comp)"  n_bits=10  bin_pt=9  preci_type=Single  exp_width=8  frac_width=24  assert_rate=off  rate_source=Explicitly  period=1  output_port=on  block_type=assert
  assextra_timestamp : xbsIndex_r4/Assert  assert_type=on  type_source=Explicitly  gui_display_data_type=Fixed-point  arith_type=Unsigned  n_bits=32  bin_pt=0  preci_type=Single  exp_width=8  frac_width=24  assert_rate=off  rate_source=Explicitly  period=1  output_port=on  block_type=assert
  buscreate : Subsystem  AncestorBlock=casper_library_flow_control/bus_create  mask(bus_create){inputNum=8}
      mask prompts: inputNum "Number of inputs:"
      mask init:
      | bus_create_init(gcb,...
      |     'inputNum', inputNum);
  extra_delay : Subsystem  AncestorBlock=casper_library_delays/pipeline  mask(pipeline){csp_latency=2}
      mask prompts: csp_latency "Latency"
      mask help:
      | An explicitly laid-out delay line to avoid mapping to SRL16s
      | for use in pipelining to help achieve timing closure.
      mask init:
      | pipeline_init(gcb,'latency',csp_latency);
      settings: AttributesFormatString=Latency = %<latency>
      mask Display:
      | port_label('input', 1, 'd');
      | port_label('output', 1, 'q');
      | disp(['Z^-', num2str(csp_latency)]);
  extracast : xbsIndex_r4/Convert  gui_display_data_type=Fixed-point  arith_type=Unsigned  n_bits=32  bin_pt=0  float_type=Single  exp_bits=8  fraction_bits=24  quantization=Truncate  overflow=Wrap  en=off  latency=1  pipeline=off  dbl_ovrd=off  block_type=convert
  extracreate : Subsystem  AncestorBlock=casper_library_flow_control/bus_create  mask(bus_create){inputNum=1}
      mask prompts: inputNum "Number of inputs:"
      mask init:
      | bus_create_init(gcb,...
      |     'inputNum', inputNum);
  io_delay : Subsystem  AncestorBlock=casper_library_delays/pipeline  mask(pipeline){csp_latency=2}
      mask prompts: csp_latency "Latency"
      mask help:
      | An explicitly laid-out delay line to avoid mapping to SRL16s
      | for use in pipelining to help achieve timing closure.
      mask init:
      | pipeline_init(gcb,'latency',csp_latency);
      settings: AttributesFormatString=Latency = %<latency>
      mask Display:
      | port_label('input', 1, 'd');
      | port_label('output', 1, 'q');
      | disp(['Z^-', num2str(csp_latency)]);
  ss : Subsystem  Tag=casper:snapshot  AncestorBlock=casper_library_scopes/snapshot  mask(snapshot){storage=bram, dram_dimm=2, dram_clock=250, nsamples=8, data_width=128, offset=off, circap=on, value=on, ext_arm=off, ext_circ=off, provide_outputs=off, use_dsp48=on}
      mask prompts: storage "Storage medium"; dram_dimm "DRAM dimm"; dram_clock "DRAM clock rate"; nsamples "Number of Samples (2^?)"; data_width "Data width"; offset "Start delay support"; circap "Circular capture support"; value "Extra value capture support"; ext_arm "External arm support"; ext_circ "External circular capture support"; provide_outputs "Provide outputs"; use_dsp48 "Use DSP48s to implement counters"
      mask help:
      | Standard snap block, but with the following optional extras;
      |  1) Optionally delay the fabric trigger by a user-specified number of valids.
      |  2) Capture continuously after a trigger until a stop pulse is received. Data is captured into BRAM continuously, with old data being overwritten until a stop command is received. Then stop capturing when memory is filled. This enables you to get some data before and some data after the stop pulse. Use the 'tr_en_cnt' register to determine where you are in your vector. 'Addr' register's MSb now indicates 'busy capturing'.
      |  3) Optionally capture a value on an input port to a register at the same time as the first data sample.
      |  4) Implement counters using DSP48Es to save resources.
      mask init: same as s_c107m32k_vlbi/snap_acc/ss
      settings: AttributesFormatString=|
      | 128 wide, 256 deep
      | debugID: 56926971
      mask TypeOptions storage: bram | dram
      mask Callback storage: snapshot_callback();
      mask TypeOptions dram_dimm: 1 | 2 | 3 | 4
      mask TypeOptions dram_clock: 200 | 250 | 266 | 300 | 333
      mask TypeOptions data_width: 8 | 16 | 32 | 64 | 128
  stop_delay : Subsystem  AncestorBlock=casper_library_delays/pipeline  mask(pipeline){csp_latency=2}
      mask prompts: csp_latency "Latency"
      mask help:
      | An explicitly laid-out delay line to avoid mapping to SRL16s
      | for use in pipelining to help achieve timing closure.
      mask init:
      | pipeline_init(gcb,'latency',csp_latency);
      settings: AttributesFormatString=Latency = %<latency>
      mask Display:
      | port_label('input', 1, 'd');
      | port_label('output', 1, 'q');
      | disp(['Z^-', num2str(csp_latency)]);
  trig_delay : Subsystem  AncestorBlock=casper_library_delays/pipeline  mask(pipeline){csp_latency=2}
      mask prompts: csp_latency "Latency"
      mask help:
      | An explicitly laid-out delay line to avoid mapping to SRL16s
      | for use in pipelining to help achieve timing closure.
      mask init:
      | pipeline_init(gcb,'latency',csp_latency);
      settings: AttributesFormatString=Latency = %<latency>
      mask Display:
      | port_label('input', 1, 'd');
      | port_label('output', 1, 'q');
      | disp(['Z^-', num2str(csp_latency)]);
  we_delay : Subsystem  AncestorBlock=casper_library_delays/pipeline  mask(pipeline){csp_latency=2}
      mask prompts: csp_latency "Latency"
      mask help:
      | An explicitly laid-out delay line to avoid mapping to SRL16s
      | for use in pipelining to help achieve timing closure.
      mask init:
      | pipeline_init(gcb,'latency',csp_latency);
      settings: AttributesFormatString=Latency = %<latency>
      mask Display:
      | port_label('input', 1, 'd');
      | port_label('output', 1, 'q');
      | disp(['Z^-', num2str(csp_latency)]);
  arm_out : Outport
  wires:
  ss/1(arm_out) -> arm_out/1
  buscreate/1(bus_out) -> io_delay/1(d)
  io_delay/1(q) -> ss/1(din)
  in_p1_d0/1 -> assert_p1_d0/1
  assert_p1_d0/1 -> buscreate/1(in1)
  in_p1_d1/1 -> assert_p1_d1/1
  assert_p1_d1/1 -> buscreate/2(in2)
  in_p1_d2/1 -> assert_p1_d2/1
  assert_p1_d2/1 -> buscreate/3(in3)
  in_p1_d3/1 -> assert_p1_d3/1
  assert_p1_d3/1 -> buscreate/4(in4)
  in_p1_d4/1 -> assert_p1_d4/1
  assert_p1_d4/1 -> buscreate/5(in5)
  in_p1_d5/1 -> assert_p1_d5/1
  assert_p1_d5/1 -> buscreate/6(in6)
  in_p1_d6/1 -> assert_p1_d6/1
  assert_p1_d6/1 -> buscreate/7(in7)
  in_p1_d7/1 -> assert_p1_d7/1
  assert_p1_d7/1 -> buscreate/8(in8)
  we/1 -> we_delay/1(d)
  we_delay/1(q) -> ss/2(we)
  trig/1 -> trig_delay/1(d)
  trig_delay/1(q) -> ss/3(trig)
  stop/1 -> stop_delay/1(d)
  stop_delay/1(q) -> ss/4(stop)
  extracreate/1(bus_out) -> extra_delay/1(d)
  extra_delay/1(q) -> extracast/1
  extracast/1 -> ss/5(vin)
  extra_timestamp/1 -> assextra_timestamp/1
  assextra_timestamp/1 -> extracreate/1(in1)
